simulink model "State_flow_GS"  (R2024a)
settings: Solver=VariableStepAuto  StartTime=0.0  StopTime=20  MaxStep=0.01  RelTol=1e-3
values from neighbouring files (symbols this model uses):
  A1 = calcolaA(k_sf_min,k_sr_min)    [controlloH2Robusto.m]    (also in controlloHinfLPV.m; state_flow.m = calcolaAssetto(k_sf_confort,k_sr_confort,c_sf_confort,c_sr_c)
  A2 = calcolaA(k_sf_min,k_sr_max)    [controlloH2Robusto.m]    (also in controlloHinfLPV.m; state_flow.m = calcolaAssetto(k_sf_normal,k_sr_normal,c_sf_normal,c_sr_norm)
  A3 = calcolaA(k_sf_max,k_sr_max)    [controlloH2Robusto.m]    (also in controlloHinfLPV.m; state_flow.m = calcolaAssetto(k_sf_sport,k_sr_sport,c_sf_sport,c_sr_sport))
  B = {B1, B2, B3, B4}    [HinfLPV_Regulation.m]    (also in L1LPV_Regulation.m; L1_H2_Hinf_dosso.m = [; L1_H2_Hinf_strada_dissestata.m = [; controlloH2H8_H8alfa.m = [)
  C = [1 0 0 0 0 0 0 0 ... (first row only)    [L1_H2_Hinf_dosso.m]    (also in L1_H2_Hinf_strada_dissestata.m; controlloH2H8_H8alfa.m; controlloH2Robusto.m = eye(8); controlloH2_dinamico.m = [)
  D = [ ... (first row only)    [controlloH2H8_H8alfa.m]    (also in controlloH2Robusto.m = zeros(8,4); controlloH2_dinamico.m = zeros(4,2); controlloH8_dinamico.m = zeros(4,2); controlloHinfLPV.m = zeros(8,4))
  E = [ ... (first row only)    [L1_H2_Hinf_dosso.m]    (also in L1_H2_Hinf_strada_dissestata.m; controlloH2H8_H8alfa.m; controlloH2Robusto.m; controlloH2_dinamico.m)
  k1 = H2H8_Regulation(A1,B,E,C22,D22,D11)    [state_flow.m]
  k2 = H2H8_Regulation(A2,B,E,C22,D22,D11)    [state_flow.m]
  k3 = H2H8_Regulation(A3,B,E,C22,D22,D11)    [state_flow.m]
  x0 = zeros(8,1)    [L1_H2_Hinf_dosso.m]    (also in L1_H2_Hinf_strada_dissestata.m; controlloH2H8_H8alfa.m; controlloH2Robusto.m; controlloH2_dinamico.m)
settings Model: Creator=alest  LastModifiedBy=alest

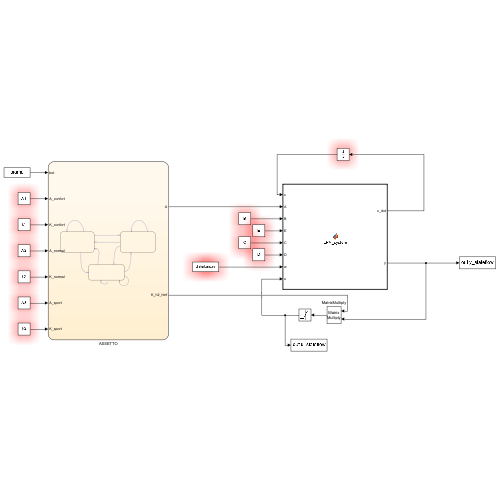
[thumbnail: Simulink's stored preview of the top-level diagram]
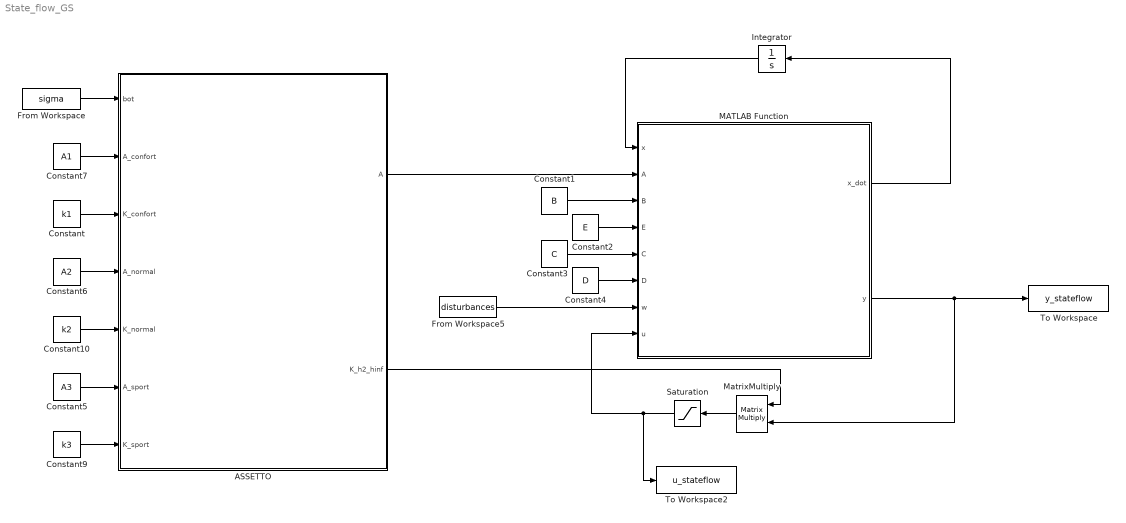
== system State_flow_GS ==
  ASSETTO : Stateflow chart  TreatAsAtomicUnit=on
  Constant : Constant  Value=k1
  Constant1 : Constant  Value=B
  Constant10 : Constant  Value=k2
  Constant2 : Constant  Value=E
  Constant3 : Constant  Value=C
  Constant4 : Constant  Value=D
  Constant5 : Constant  Value=A3
  Constant6 : Constant  Value=A2
  Constant7 : Constant  Value=A1
  Constant9 : Constant  Value=k3
  From Workspace : FromWorkspace  VariableName=sigma
  From Workspace5 : FromWorkspace  VariableName=disturbances  OutputAfterFinalValue=Holding final value
  Integrator : Integrator  InitialCondition=x0
  MATLAB Function : MATLAB Function  TreatAsAtomicUnit=on
  MatrixMultiply : Product  Multiplication=Matrix(*)
  Saturation : Saturate  UpperLimit=4000  LowerLimit=-4000
  To Workspace : ToWorkspace  VariableName=y_stateflow  SaveFormat=Timeseries  SampleTime=-1
  To Workspace2 : ToWorkspace  VariableName=u_stateflow  SaveFormat=Timeseries  SampleTime=-1
  wires:
  Constant4/1 -> MATLAB Function/6(D)
  MATLAB Function/2(y) -> MatrixMultiply/2, To Workspace/1
  From Workspace5/1 -> MATLAB Function/7(w)
  Constant3/1 -> MATLAB Function/5(C)
  Constant2/1 -> MATLAB Function/4(E)
  Constant1/1 -> MATLAB Function/3(B)
  MATLAB Function/1(x_dot) -> Integrator/1
  Integrator/1 -> MATLAB Function/1(x)
  Constant5/1 -> ASSETTO/6(A_sport)
  Constant6/1 -> ASSETTO/4(A_normal)
  Constant7/1 -> ASSETTO/2(A_confort)
  Constant/1 -> ASSETTO/3(K_confort)
  Constant10/1 -> ASSETTO/5(K_normal)
  Constant9/1 -> ASSETTO/7(K_sport)
  ASSETTO/1(A) -> MATLAB Function/2(A)
  ASSETTO/2(K_h2_hinf) -> MatrixMultiply/1
  From Workspace/1 -> ASSETTO/1(bot)
  MatrixMultiply/1 -> Saturation/1
  Saturation/1 -> To Workspace2/1, MATLAB Function/8(u)

== matlab function State_flow_GS/MATLAB Function ==
  data: x_dot output; x input; A input; y output; B input; E input; C input; D input; w input; u input
function [x_dot,y] = LPV_system(x,A,B,E,C,D,w,u)

x_dot=A*x+B*u+E*w;

y = C*x;

end

== stateflow chart State_flow_GS/ASSETTO ==
  state sport
    entry:K_h2_hinf=K_sport;
    entry:A=A_sport;
  state confort
    entry:K_h2_hinf=K_confort;
    entry:A=A_confort;
  state normal
    entry:K_h2_hinf=K_normal;
    entry:A=A_normal;
  sport -> sport [order 3] : [bot==2]
  confort -> confort [order 3] : [bot==1]
  sport -> confort [order 2] : [bot==1]
  confort -> sport [order 1] : [bot==2]
  confort -> normal [order 2] : [bot==0]
  normal -> sport [order 2] : [bot==2]
  sport -> normal [order 1] : [bot==0]
  normal -> confort [order 1] : [bot==1]
  normal -> normal [order 3] : [bot==0]
  (default) -> normal
  data: bot input; A_confort input; K_confort input; A_normal input; K_normal input; A_sport input; A output size=[8 8]; K_h2_hinf output size=[2 8]; K_sport input
